simulink model "tanque"  (R2025b)
settings: Solver=VariableStepAuto  StartTime=0.0  StopTime=10.0  RelTol=1e-3
values from neighbouring files (symbols this model uses):
  ae0 = 0.6    [Aula08_lab.m]    (also in Lab10.m; Lab5_6.m; lab3.m; lab4.m = 0:0.01:1)
  as0 = 0.5    [Aula08_lab.m]    (also in Lab10.m; Lab5_6.m; lab3.m; lab4.m = 0:0.01:1)

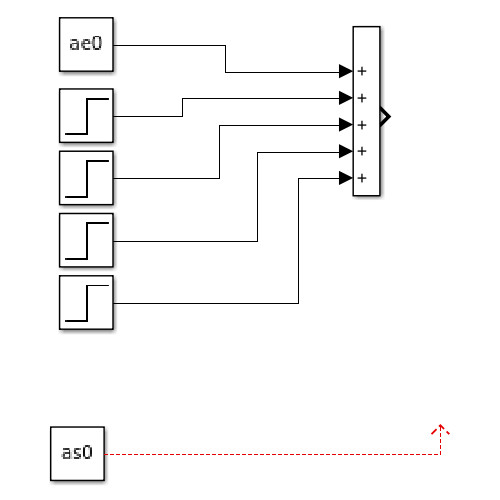
[thumbnail: Simulink's stored preview of the top-level diagram]
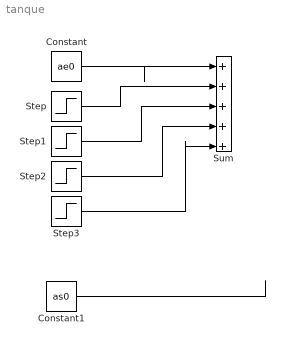
== system tanque ==
  Constant : Constant  Value=ae0
  Constant1 : Constant  Value=as0
  Step{,1..3} (4 alike) : Step  SampleTime=0
  Sum : Sum  Inputs=|+++++
  wires:
  Constant/1 -> Sum/1
  Step/1 -> Sum/2
  Step1/1 -> Sum/3
  Step2/1 -> Sum/4
  Step3/1 -> Sum/5
  Constant1/1 -> ?
